simulink model "EspacoDeEstados"  (R2026a)
settings: Solver=VariableStepAuto
values from neighbouring files (symbols this model uses):
  A = [0,           1,          0 ... (first row only)    [paramEmc.m]
  B = [0 ... (first row only)    [paramEmc.m]
  C = eye(3)    [paramEmc.m]
  x0 = [deg2rad(12); 0; 0]    [paramEmc.m]
undefined symbols (not defined in the file or in its folder): K
settings Model: Creator=Agmar  LastModifiedBy=Enzo

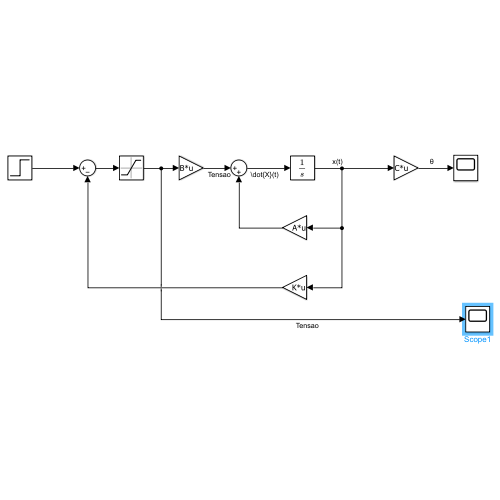
[thumbnail: Simulink's stored preview of the top-level diagram]
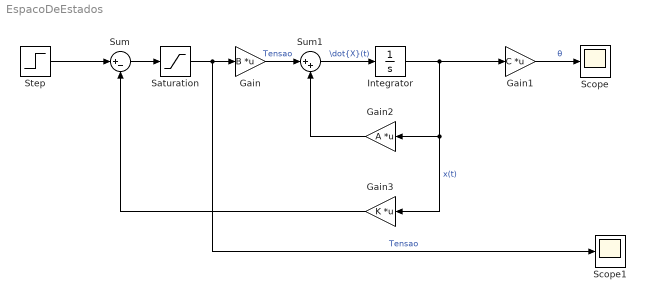
== system EspacoDeEstados ==
  Gain : Gain  Gain=B  Multiplication=Matrix(K*u)
  Gain1 : Gain  Gain=C  Multiplication=Matrix(K*u)
  Gain2 : Gain  Gain=A  Multiplication=Matrix(K*u)
  Gain3 : Gain  Gain=K  Multiplication=Matrix(K*u)
  Integrator : Integrator  InitialCondition=x0
  Saturation : Saturate  UpperLimit=24  LowerLimit=-24
  Scope : Scope
      settings: ActiveDisplayYMinimum=-0.088484185054417033  ActiveDisplayYMaximum=0.29872046500604632
  Scope1 : Scope
      settings: ActiveDisplayYMinimum=-2.0430899787683976  ActiveDisplayYMaximum=18.272124349762631
  Step : Step  Time=0  FinalValue=0  SampleTime=0
  Sum : Sum  Inputs=|+-
  Sum1 : Sum  Inputs=|++
  wires:
  Step/1 -> Sum/1
  Sum1/1 -> Integrator/1  "\\dot{X}(t)"
  Gain/1 -> Sum1/1  "Tensao"
  Gain2/1 -> Sum1/2
  Gain3/1 -> Sum/2
  Gain1/1 -> Scope/1  "θ"
  Integrator/1 -> Gain3/1, Gain2/1, Gain1/1  "x(t)"
  Sum/1 -> Saturation/1
  Saturation/1 -> Scope1/1, Gain/1  "Tensao"
